simulink model "Full_Car_Model"  (R2023b)
settings: Solver=FixedStepAuto  StartTime=0.0  StopTime=t_end_sim  FixedStep=Ts_sim  RelTol=1e-3
values from neighbouring files (symbols this model uses):
  a_b_ref_sat = [ zeros(1,10) ... (first row only)    [A1_Init.m]    (also in C1_MonteCarloAnalysis.m)
  adaptive = 3    [A1_Init.m]    (also in C1_MonteCarloAnalysis.m = 1)
  data = A2_Full_car_model_parameters_4onBoard()    [A1_Init.m]    (also in C1_MonteCarloAnalysis.m)
  Ft_demand_F = [zeros(1,601) 200*ones(1,2400)]./data.R_F    [A1_Init.m]    (also in C1_MonteCarloAnalysis.m)
  Ft_demand_R = [zeros(1,(601-length(l_discr)))              200*ones(1,(2400+length(l_discr)))]./data.R_R    [A1_Init.m]    (also in C1_MonteCarloAnalysis.m)
  handmade_front = strcat(currentPath,'\Road_profiles\height_crg_files\','handmade_step_3cm_singlefunctions.crg')    [A1_Init.m]    (also in C1_MonteCarloAnalysis.m)
  handmade_mu_front = strcat(currentPath,'\Road_profiles\friction_crg_files\','handmade_fric_step_01_singlefunctions.crg')    [A1_Init.m]    (also in C1_MonteCarloAnalysis.m)
  handmade_mu_rear = handmade_mu_front    [A1_Init.m]    (also in C1_MonteCarloAnalysis.m)
  handmade_rear = handmade_front    [A1_Init.m]    (also in C1_MonteCarloAnalysis.m)
  LowLim_Q1 = -10    [A1_Init.m]    (also in C1_MonteCarloAnalysis.m)
  M = N    (= 10)    [A1_Init.m]    (also in C1_MonteCarloAnalysis.m)
  mu_distance = test_distance    [A1_Init.m]    (also in C1_MonteCarloAnalysis.m)
  mu_road = [ones(1,1001), 0.1*ones(1,2000)]    [A1_Init.m]    (also in C1_MonteCarloAnalysis.m)
  N = 10    [A1_Init.m]    (also in C1_MonteCarloAnalysis.m)
  N_iter = 3    [A1_Init.m]    (also in C1_MonteCarloAnalysis.m)
  omega_ini_F_L = x_u_dot_ini_F_L/data.R_F    [A1_Init.m]    (also in C1_MonteCarloAnalysis.m)
  omega_ini_F_R = x_u_dot_ini_R_R/data.R_F    [A1_Init.m]    (also in C1_MonteCarloAnalysis.m)
  omega_ini_R_L = x_u_dot_ini_R_L/data.R_R +2.483*1e-6    [A1_Init.m]    (also in C1_MonteCarloAnalysis.m)
  omega_ini_R_R = x_u_dot_ini_R_R/data.R_R+2.483*1e-6    [A1_Init.m]    (also in C1_MonteCarloAnalysis.m)
  passive = 2    [A1_Init.m]    (also in C1_MonteCarloAnalysis.m)
  Pitch = 0    [A1_Init.m]    (also in C1_MonteCarloAnalysis.m)
  Pitch_dot = 0    [A1_Init.m]    (also in C1_MonteCarloAnalysis.m)
  preview = 2    [A1_Init.m]    (also in C1_MonteCarloAnalysis.m)
  Q1 = 1e6    (= 1000000)    [A1_Init.m]    (also in C1_MonteCarloAnalysis.m)
  Q1_sat = 0    [A1_Init.m]    (also in C1_MonteCarloAnalysis.m)
  Q2 = 1e5    (= 100000)    [A1_Init.m]    (also in C1_MonteCarloAnalysis.m)
  QN1 = 0    [A1_Init.m]    (also in C1_MonteCarloAnalysis.m)
  QN2 = 0    [A1_Init.m]    (also in C1_MonteCarloAnalysis.m)
  R1 = 1e10    (= 10000000000)    [A1_Init.m]    (also in C1_MonteCarloAnalysis.m)
  r1_h0 = 0.99    [A1_Init.m]    (also in C1_MonteCarloAnalysis.m)
  r1_k = 1000    [A1_Init.m]    (also in C1_MonteCarloAnalysis.m)
  r1_max = 11    [A1_Init.m]    (also in C1_MonteCarloAnalysis.m)
  r1_min = -10    [A1_Init.m]    (also in C1_MonteCarloAnalysis.m)
  r2 = 2    [A1_Init.m]    (also in C1_MonteCarloAnalysis.m)
  R2 = 1e2    (= 100)    [A1_Init.m]    (also in C1_MonteCarloAnalysis.m)
  R2_rl = 2    [A1_Init.m]    (also in C1_MonteCarloAnalysis.m)
  road_profile = [zeros(1,801),ones(1,2200)*10*Step_selector]    [A1_Init.m]    (also in C1_MonteCarloAnalysis.m)
  T_distance = test_distance    [A1_Init.m]    (also in C1_MonteCarloAnalysis.m)
  T_hs_ini_F_L = 0    [A1_Init.m]    (also in C1_MonteCarloAnalysis.m)
  T_hs_ini_F_R = 0    [A1_Init.m]    (also in C1_MonteCarloAnalysis.m)
  T_hs_ini_R_L = 0    [A1_Init.m]    (also in C1_MonteCarloAnalysis.m)
  T_hs_ini_R_R = 0    [A1_Init.m]    (also in C1_MonteCarloAnalysis.m)
  test_distance = 0:0.01:30    [A1_Init.m]    (also in C1_MonteCarloAnalysis.m)
  theta_s_ini_F_L = 0    [A1_Init.m]    (also in C1_MonteCarloAnalysis.m)
  theta_s_ini_F_R = 0    [A1_Init.m]    (also in C1_MonteCarloAnalysis.m)
  theta_s_ini_R_L = 0    [A1_Init.m]    (also in C1_MonteCarloAnalysis.m)
  theta_s_ini_R_R = 0    [A1_Init.m]    (also in C1_MonteCarloAnalysis.m)
  theta_w_ini_F_L = -1.056*1e-2    (= -0.01056)    [A1_Init.m]    (also in C1_MonteCarloAnalysis.m)
  theta_w_ini_R_L = -1.056*1e-2    (= -0.01056)    [A1_Init.m]    (also in C1_MonteCarloAnalysis.m)
  Ts = 1e-3*[0 5 10 15 20 25 30 40 60 80 100]    [A1_Init.m]    (also in C1_MonteCarloAnalysis.m)
  w1_h0 = 0.0008    [A1_Init.m]    (also in C1_MonteCarloAnalysis.m)
  w1_k = 5000    [A1_Init.m]    (also in C1_MonteCarloAnalysis.m)
  w1_max = 9    [A1_Init.m]    (also in C1_MonteCarloAnalysis.m)
  w1_min = -10    [A1_Init.m]    (also in C1_MonteCarloAnalysis.m)
  w1_sat = 0.085    [A1_Init.m]    (also in C1_MonteCarloAnalysis.m)
  w2_h0 = 2    [A1_Init.m]    (also in C1_MonteCarloAnalysis.m)
  w2_inc = 0.05    [A1_Init.m]    (also in C1_MonteCarloAnalysis.m)
  w2_k = 10    [A1_Init.m]    (also in C1_MonteCarloAnalysis.m)
  w2_max = 5.3    [A1_Init.m]    (also in C1_MonteCarloAnalysis.m)
  w2_min = -10    [A1_Init.m]    (also in C1_MonteCarloAnalysis.m)
  Wmat_NMPC_init = [W(1,:) W(2,:) W(3,:) W(4,:)]    [A1_Init.m]    (also in C1_MonteCarloAnalysis.m)
  WNmat_NMPC_init = [WN(1,:) WN(2,:)]    [A1_Init.m]    (also in C1_MonteCarloAnalysis.m)
  X_0 = [z_b_dot_ini z_b_ini z_u_dot_ini_F_L z_u_ini_F_L x_b_dot_ini x_b_ini x_u_dot_ini_F_L x_u_ini_F_L          omega_ini_F_L theta_w_ini_F_L omega_ini_F_L theta_s_ini_F_L torque_ini_F_L]    [A1_Init.m]    (also in C1_MonteCarloAnalysis.m)
  x_b_dot_ini = speed_ini/3.6    (= 11.1111111111)    [A1_Init.m]    (also in C1_MonteCarloAnalysis.m)
  x_b_ini = data.b+pos_ini    [A1_Init.m]    (also in C1_MonteCarloAnalysis.m)
  x_u_dot_ini_F_L = speed_ini/3.6 - 1.125*1e-4    (= 11.1109986111)    [A1_Init.m]    (also in C1_MonteCarloAnalysis.m)
  x_u_dot_ini_F_R = speed_ini/3.6 - 1.125*1e-4    (= 11.1109986111)    [A1_Init.m]    (also in C1_MonteCarloAnalysis.m)
  x_u_dot_ini_R_L = speed_ini/3.6 - 1.125*1e-4    (= 11.1109986111)    [A1_Init.m]    (also in C1_MonteCarloAnalysis.m)
  x_u_dot_ini_R_R = speed_ini/3.6 - 1.125*1e-4    (= 11.1109986111)    [A1_Init.m]    (also in C1_MonteCarloAnalysis.m)
  x_u_ini_F_L = data.a+data.b+pos_ini    [A1_Init.m]    (also in C1_MonteCarloAnalysis.m)
  x_u_ini_F_R = data.a+data.b+pos_ini    [A1_Init.m]    (also in C1_MonteCarloAnalysis.m)
  x_u_ini_R_L = pos_ini    (= 0)    [A1_Init.m]    (also in C1_MonteCarloAnalysis.m)
  x_u_ini_R_R = pos_ini    (= 0)    [A1_Init.m]    (also in C1_MonteCarloAnalysis.m)
  z_b_dot_ini = 0    [A1_Init.m]    (also in C1_MonteCarloAnalysis.m)
  z_b_ini = 0    [A1_Init.m]    (also in C1_MonteCarloAnalysis.m)
  z_u_dot_ini_F_L = 0    [A1_Init.m]    (also in C1_MonteCarloAnalysis.m)
  z_u_dot_ini_F_R = 0    [A1_Init.m]    (also in C1_MonteCarloAnalysis.m)
  z_u_dot_ini_R_L = 0    [A1_Init.m]    (also in C1_MonteCarloAnalysis.m)
  z_u_dot_ini_R_R = 0    [A1_Init.m]    (also in C1_MonteCarloAnalysis.m)
  z_u_ini_F_L = 0    [A1_Init.m]    (also in C1_MonteCarloAnalysis.m)
  z_u_ini_F_R = 0    [A1_Init.m]    (also in C1_MonteCarloAnalysis.m)
  z_u_ini_R_L = 0    [A1_Init.m]    (also in C1_MonteCarloAnalysis.m)
  z_u_ini_R_R = 0    [A1_Init.m]    (also in C1_MonteCarloAnalysis.m)
undefined symbols (not defined in the file or in its folder): Delay_step, road_with_noise
libraries: mfswift_library x8, rllib x4, simulink x4
(part 1 of 7)
settings Model: Creator=victor  LastModifiedBy=d106370
settings SolverCC: AlgebraicLoopSolver=TrustRegion
settings DataIOCC: SaveOutput=off  SignalLogging=off  DSMLogging=off  SaveTime=off  ReturnWorkspaceOutputs=off
settings DebuggingCC: UnconnectedInputMsg=warning  UnconnectedOutputMsg=warning  UnconnectedLineMsg=warning
settings ModelReferenceCC: EnableRefExpFcnMdlSchedulingChecks=on
settings SFSimCC: CustomCodeUndefinedFunction=UseInterfaceOnly
settings RTWCC: DLArmComputeVersion=19.05

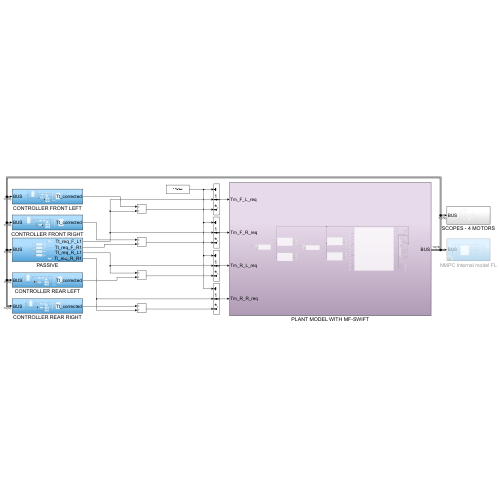
[thumbnail: Simulink's stored preview of the top-level diagram]
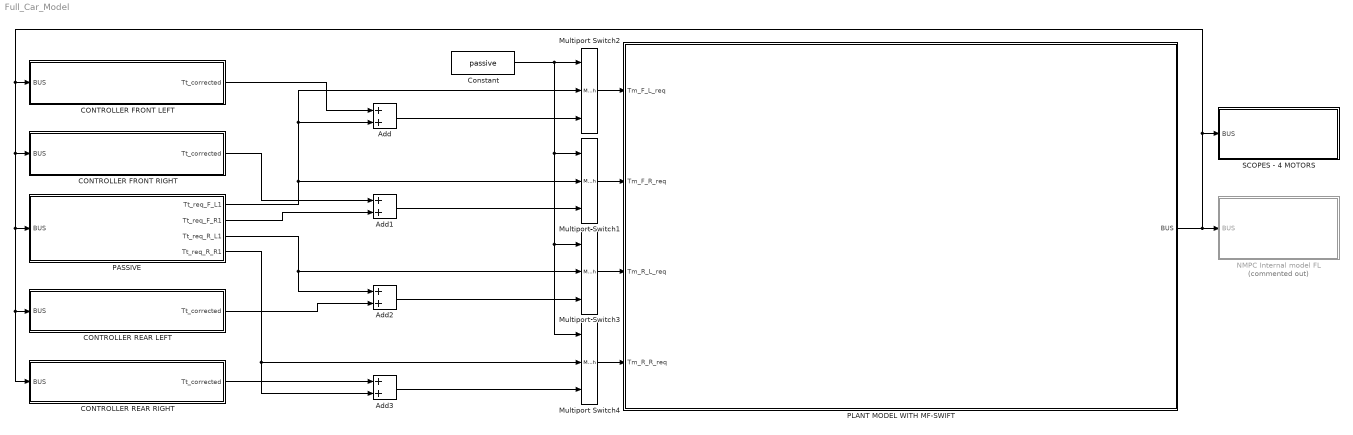
== system Full_Car_Model ==
  Add{,1..3} (4 alike) : Sum
  CONTROLLER FRONT LEFT : Subsystem
  CONTROLLER FRONT RIGHT : Subsystem
  CONTROLLER REAR LEFT : Subsystem
  CONTROLLER REAR RIGHT : Subsystem
  Constant : Constant  Value=passive
  Multiport Switch{1..4} (4 alike) : MultiPortSwitch  Inputs=2  SaturateOnIntegerOverflow=off  InputSameDT=off
  NMPC Internal model FL : Subsystem  Commented=on
  PASSIVE : Subsystem
  PLANT MODEL WITH MF-SWIFT : Subsystem
  SCOPES - 4 MOTORS : Subsystem
  wires:
  Add3/1 -> Multiport Switch4/3
  Multiport Switch4/1 -> PLANT MODEL WITH MF-SWIFT/4(Tm_R_R_req)
  Multiport Switch2/1 -> PLANT MODEL WITH MF-SWIFT/1(Tm_F_L_req)
  CONTROLLER REAR LEFT/1(Tt_corrected) -> Add2/2
  Multiport Switch1/1 -> PLANT MODEL WITH MF-SWIFT/2(Tm_F_R_req)
  PASSIVE/2(Tt_req_F_R1) -> Add1/2
  CONTROLLER FRONT RIGHT/1(Tt_corrected) -> Add1/1
  CONTROLLER FRONT LEFT/1(Tt_corrected) -> Add/1
  PASSIVE/1(Tt_req_F_L1) -> Multiport Switch1/2, Multiport Switch2/2, Add/2
  Add2/1 -> Multiport Switch3/3
  Add/1 -> Multiport Switch2/3
  PLANT MODEL WITH MF-SWIFT/1(BUS) -> CONTROLLER FRONT LEFT/1(BUS), CONTROLLER REAR RIGHT/1(BUS), CONTROLLER REAR LEFT/1(BUS), PASSIVE/1(BUS), CONTROLLER FRONT RIGHT/1(BUS), SCOPES - 4 MOTORS/1(BUS), NMPC Internal model FL/1(BUS)
  Add1/1 -> Multiport Switch1/3
  CONTROLLER REAR RIGHT/1(Tt_corrected) -> Add3/1
  PASSIVE/3(Tt_req_R_L1) -> Add2/1, Multiport Switch3/2
  Constant/1 -> Multiport Switch4/1, Multiport Switch3/1, Multiport Switch1/1, Multiport Switch2/1
  Multiport Switch3/1 -> PLANT MODEL WITH MF-SWIFT/3(Tm_R_L_req)
  PASSIVE/4(Tt_req_R_R1) -> Multiport Switch4/2, Add3/2

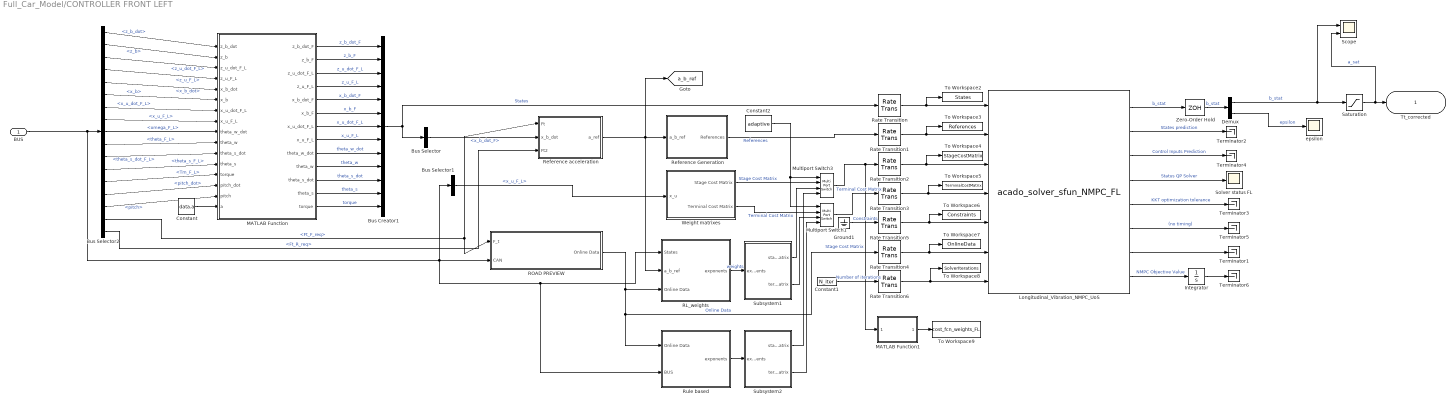
== system Full_Car_Model/CONTROLLER FRONT LEFT ==
  BUS : Inport
  Bus Creator1 : BusCreator  Inputs=13
  Bus Selector : BusSelector  OutputSignals=x_b_dot_F
  Bus Selector1 : BusSelector  OutputSignals=States.x_u_F_L
  Bus Selector2 : BusSelector  OutputSignals=States.z_b_dot,States.z_b,States.z_u_dot_F_L,States.z_u_F_L,States.x_b_dot,States.x_b,States.x_u_dot_F_L,States.x_u_F_L,States.omega_F_L,States.theta_F_L,Differentials.theta_s_dot_F_L,Differentials.theta_s_F_L,Traction_forces.Tm_F_L,States.pitch_dot,States.pitch,Traction_forces.Ft_F_req,Traction_forces.Ft_R_req
  Constant : Constant  Value=data.a
  Constant1 : Constant  Value=N_iter
  Constant2 : Constant  Value=adaptive
  Demux : Demux  Outputs=2
  Ground1 : Ground
  Integrator : Integrator
  Longitudinal_Vibration_NMPC_UoS : S-Function  FunctionName=acado_solver_sfun_NMPC_FL  Parameters=xInit, zInit, uInit, Wmat_NMPC_init, WNmat_NMPC_init, bValues  SFunctionDeploymentMode=off  EnableBusSupport=off  mask(Legacy Function){SFunctionSpec=acado_step(ACADOinput u1[1], ACADOoutput y1[1]), ShowSpec=on}
      mask prompts: ShowSpec "Display function specification"
      mask help:
      | This block allows you to call the legacy functions specified by the following Legacy Code Tool definition:
      | def.SFunctionName = 'acado_solver_sfun';
      | def.OutputFcnSpec = 'acado_step(ACADOinput u1[1], ACADOoutput y1[1])';
      | def.StartFcnSpec = 'acado_initialize( void )';
      | def.TerminateFcnSpec = 'acado_cleanup( void )';
      | def.HeaderFiles = {'acado_common.h', 'acado_solver_sfunction.h'};
      | def.SourceFiles = {'acado_solver.c', 'acado_integrator.c', 'acado_auxiliary_functions.c', 'acado_solver_sfunction.c', 'acado_qpoases_interface.cpp', 'qpoases/SRC/Bounds.cpp', 'qpoases/SRC/Constraints.cpp', 'qpoases/SRC/CyclingManager.cpp', 'qpoases/SRC/Indexlist.cpp', 'qpoases/SRC/MessageHandling.cpp', 'qpoases/SRC/QProblem.cpp', 'qpoases/SRC/QProblemB.cpp', 'qpoases/SRC/SubjectTo.cpp', 'qpoases/SRC/Utils.cpp', 'qpoases/SRC/EXTRAS/SolutionAnalysis.cpp'};
      | def.IncPaths = {'qpoases', 'qpoases/INCLUDE', 'qpoases/SRC'};
      | def.Options.language = 'C++';
      mask Help: <p>This block was generated automatically by the Legacy Code Tool. For detailed help on this tool, call<a href="matlab:legacy_code('help')"> legacy_code('help')</a>.</p>
      mask Callback ShowSpec:
      | if strcmp(get_param(gcbh, 'ShowSpec'), 'on')
      |   set_param(gcbh, 'MaskDisplay', sprintf('fprintf(''%s'');', get_param(gcbh, 'SFunctionSpec')));
      | else
      |   set_param(gcbh, 'MaskDisplay', sprintf('fprintf(''%s'');', get_param(gcbh, 'FunctionName')));
      | end
      mask Display: fprintf('acado_step(ACADOinput u1[1], ACADOoutput y1[1])');
  MATLAB Function : MATLAB Function  TreatAsAtomicUnit=on
  MATLAB Function1 : MATLAB Function  TreatAsAtomicUnit=on
  Multiport Switch1 : MultiPortSwitch  SaturateOnIntegerOverflow=off  InputSameDT=off
  Multiport Switch3 : MultiPortSwitch  SaturateOnIntegerOverflow=off  InputSameDT=off
  RL_weights : Subsystem
  ROAD PREVIEW : Subsystem
  Rate Transition : RateTransition  InitialCondition=X_0  OutPortSampleTime=Ts(2)
  Rate Transition{1,4..6} (4 alike) : RateTransition  OutPortSampleTime=Ts(2)
  Rate Transition2 : RateTransition  InitialCondition=Wmat_NMPC_init  OutPortSampleTime=Ts(2)
  Rate Transition3 : RateTransition  InitialCondition=WNmat_NMPC_init  OutPortSampleTime=Ts(2)
  Reference Generation : MATLAB Function  TreatAsAtomicUnit=on
  Reference acceleration : Subsystem
  Rule based : Subsystem
  Saturation : Saturate  UpperLimit=data.Ub_Tm  LowerLimit=data.Lb_Tm
  Scope : Scope  NumInputPorts=2
  Solver status FL : Scope
  Subsystem1 : Subsystem
  Subsystem2 : Subsystem
  Terminator{1..6} (6 alike) : Terminator
  To Workspace2 : ToWorkspace  VariableName=States  SaveFormat=Timeseries  SampleTime=-1
  To Workspace3 : ToWorkspace  VariableName=References  SaveFormat=Timeseries  SampleTime=-1
  To Workspace4 : ToWorkspace  VariableName=StageCostMatrix  SaveFormat=Timeseries  SampleTime=-1
  To Workspace5 : ToWorkspace  VariableName=TerminalCostMatrix  SaveFormat=Timeseries  SampleTime=-1
  To Workspace6 : ToWorkspace  VariableName=Constraints  SaveFormat=Timeseries  SampleTime=-1
  To Workspace7 : ToWorkspace  VariableName=OnlineData  SaveFormat=Timeseries  SampleTime=-1
  To Workspace8 : ToWorkspace  VariableName=SolverIterations  SaveFormat=Timeseries  SampleTime=-1
  To Workspace9 : ToWorkspace  VariableName=cost_fcn_weights_FL  SaveFormat=Timeseries  SampleTime=-1
  Weight matrixes : Subsystem
  Zero-Order Hold : ZeroOrderHold  SampleTime=Ts(2)
  epsilon : Scope
  Tt_corrected : Outport
  tag scope: a_b_ref=global
  wires:
  Subsystem1/2(terminal cost matrix) -> Multiport Switch1/3
  Saturation/1 -> Scope/2, Tt_corrected/1  "a_sat"
  MATLAB Function/8(x_u_F_L) -> Bus Creator1/8  "x_u_F_L"
  MATLAB Function/3(z_u_dot_F_L) -> Bus Creator1/3  "z_u_dot_F_L"
  Weight matrixes/1(Stage Cost Matrix) -> Multiport Switch3/2  "Stage Cost Matrix"
  MATLAB Function/1(z_b_dot_F) -> Bus Creator1/1  "z_b_dot_F"
  Constant1/1 -> Rate Transition6/1  "Number of iterations"
  MATLAB Function/2(z_b_F) -> Bus Creator1/2  "z_b_F"
  MATLAB Function/6(x_b_F) -> Bus Creator1/6  "x_b_F"
  Bus Selector2/14 -> MATLAB Function/14(pitch_dot)  "<pitch_dot>"
  MATLAB Function/7(x_u_dot_F_L) -> Bus Creator1/7  "x_u_dot_F_L"
  Longitudinal_Vibration_NMPC_UoS/2 -> Terminator2/1  "States prediction"
  Weight matrixes/2(Terminal Cost Matrix) -> Multiport Switch1/2  "Terminal Cost Matrix"
  Bus Selector2/6 -> MATLAB Function/6(x_b)  "<x_b>"
  Longitudinal_Vibration_NMPC_UoS/4 -> Solver status FL/1  "Status QP Solver"
  Reference acceleration/1(a_ref) -> Reference Generation/1(a_b_ref), [a_b_ref], RL_weights/2(a_b_ref)
  Integrator/1 -> Terminator6/1
  Bus Selector2/1 -> MATLAB Function/1(z_b_dot)  "<z_b_dot>"
  Rate Transition2/1 -> Longitudinal_Vibration_NMPC_UoS/3, To Workspace4/1
  Bus Selector2/9 -> MATLAB Function/9("theta_w_dot ")  "<omega_F_L>"
  Rate Transition4/1 -> Longitudinal_Vibration_NMPC_UoS/6, To Workspace7/1
  Bus Selector2/8 -> MATLAB Function/8("x_u_F_L ")  "<x_u_F_L>"
  BUS/1 -> Bus Selector2/1, Rule based/2(BUS), RL_weights/1(States), Bus Selector1/1, ROAD PREVIEW/2(CAN)
  Rate Transition3/1 -> Longitudinal_Vibration_NMPC_UoS/4, To Workspace5/1
  RL_weights/1(exponents) -> Subsystem1/1(exponents)  "weights"
  ROAD PREVIEW/1(Online Data) -> Rule based/1(Online Data), Rate Transition4/1, RL_weights/3(Online Data)  "Online Data"
  Bus Selector2/12 -> MATLAB Function/12("theta_s ")  "<theta_s_F_L>"
  Subsystem2/2(terminal cost matrix) -> Multiport Switch1/4
  MATLAB Function/9(theta_w_dot) -> Bus Creator1/9  "theta_w_dot"
  Multiport Switch3/1 -> Rate Transition2/1, MATLAB Function1/1(Wmat_NMPC)  "Stage Cost Matrix"
  Constant/1 -> MATLAB Function/16(a)
  Bus Selector2/2 -> MATLAB Function/2(z_b)  "<z_b>"
  Bus Selector2/11 -> MATLAB Function/11("theta_s_dot ")  "<theta_s_dot_F_L>"
  MATLAB Function/13(torque) -> Bus Creator1/13  "torque"
  Longitudinal_Vibration_NMPC_UoS/3 -> Terminator4/1  "Control Inputs Prediction"
  MATLAB Function/10(theta_w) -> Bus Creator1/10  "theta_w"
  Longitudinal_Vibration_NMPC_UoS/6 -> Terminator5/1  "(no timing)"
  Demux/2 -> epsilon/1  "epsilon"
  Rate Transition5/1 -> Longitudinal_Vibration_NMPC_UoS/5, To Workspace6/1
  MATLAB Function/11(theta_s_dot) -> Bus Creator1/11  "theta_s_dot"
  MATLAB Function/5(x_b_dot_F) -> Bus Creator1/5  "x_b_dot_F"
  Bus Selector/1 -> Reference acceleration/2(x_b_dot)  "<x_b_dot_F>"
  Longitudinal_Vibration_NMPC_UoS/7 -> Terminator1/1
  Bus Selector2/13 -> MATLAB Function/13("torque ")  "<Tm_F_L>"
  Bus Selector2/16 -> Reference acceleration/1(Ft), ROAD PREVIEW/1(F_t)  "<Ft_F_req>"
  Subsystem1/1(stage cost matrix) -> Multiport Switch3/3
  Bus Selector2/10 -> MATLAB Function/10("theta_w ")  "<theta_F_L>"
  Reference Generation/1(References) -> Rate Transition1/1  "References"
  Ground1/1 -> Rate Transition5/1  "Constraints"
  Rate Transition6/1 -> Longitudinal_Vibration_NMPC_UoS/7, To Workspace8/1
  Subsystem2/1(stage cost matrix) -> Multiport Switch3/4
  Bus Selector2/5 -> MATLAB Function/5(x_b_dot)  "<x_b_dot>"
  Bus Selector2/7 -> MATLAB Function/7("x_u_dot_F_L ")  "<x_u_dot_F_L>"
  Bus Selector2/15 -> MATLAB Function/15(pitch)  "<pitch>"
  MATLAB Function/12(theta_s) -> Bus Creator1/12  "theta_s"
  Longitudinal_Vibration_NMPC_UoS/5 -> Terminator3/1  "KKT optimization tolerance"
  Bus Creator1/1 -> Rate Transition/1, Bus Selector/1  "States"
  Rate Transition/1 -> Longitudinal_Vibration_NMPC_UoS/1, To Workspace2/1
  Bus Selector2/4 -> MATLAB Function/4("z_u_F_L ")  "<z_u_F_L>"
  Bus Selector2/17 -> Reference acceleration/3(Ft2)  "<Ft_R_req>"
  MATLAB Function/4(z_u_F_L) -> Bus Creator1/4  "z_u_F_L"
  Rate Transition1/1 -> Longitudinal_Vibration_NMPC_UoS/2, To Workspace3/1
  Multiport Switch1/1 -> Rate Transition3/1  "Terminal Cost Matrix"
  Bus Selector1/1 -> Weight matrixes/1(x_u)  "<x_u_F_L>"
  Bus Selector2/3 -> MATLAB Function/3("z_u_dot_F_L ")  "<z_u_dot_F_L>"
  Constant2/1 -> Multiport Switch3/1, Multiport Switch1/1
  Longitudinal_Vibration_NMPC_UoS/8 -> Integrator/1  "NMPC Objective Value"
  Longitudinal_Vibration_NMPC_UoS/1 -> Zero-Order Hold/1  "b_stat"
  Demux/1 -> Scope/1, Saturation/1  "b_stat"
  Zero-Order Hold/1 -> Demux/1  "b_stat"
  MATLAB Function1/1(cost_fcn_weights) -> To Workspace9/1
  Rule based/1(exponents) -> Subsystem2/1(exponents)

== system Full_Car_Model/CONTROLLER FRONT RIGHT ==
  BUS : Inport
  Bus Creator1 : BusCreator  Inputs=13
  Bus Selector : BusSelector  OutputSignals=x_b_dot_F
  Bus Selector1 : BusSelector  OutputSignals=States.x_u_F_R
  Bus Selector2 : BusSelector  OutputSignals=States.z_b_dot,States.z_b,States.z_u_dot_F_R,States.z_u_F_R,States.x_b_dot,States.x_b,States.x_u_dot_F_R,States.x_u_F_R,States.omega_F_R,States.theta_F_R,Differentials.theta_s_dot_F_R,Differentials.theta_s_F_R,Traction_forces.Tm_F_R,States.pitch_dot,States.pitch,Traction_forces.Ft_F_req,Traction_forces.Ft_R_req
  Constant : Constant  Value=data.a
  Constant1 : Constant  Value=N_iter
  Constant2 : Constant  Value=adaptive
  Demux : Demux  Outputs=2
  Ground1 : Ground
  Integrator : Integrator
  Longitudinal_Vibration_NMPC_UoS : S-Function  FunctionName=acado_solver_sfun_NMPC_FR  Parameters=xInit, zInit, uInit, Wmat_NMPC_init, WNmat_NMPC_init, bValues  SFunctionDeploymentMode=off  EnableBusSupport=off  mask(Legacy Function){SFunctionSpec=acado_step(ACADOinput u1[1], ACADOoutput y1[1]), ShowSpec=on}
      mask prompts: ShowSpec "Display function specification"
      mask help:
      | This block allows you to call the legacy functions specified by the following Legacy Code Tool definition:
      | def.SFunctionName = 'acado_solver_sfun';
      | def.OutputFcnSpec = 'acado_step(ACADOinput u1[1], ACADOoutput y1[1])';
      | def.StartFcnSpec = 'acado_initialize( void )';
      | def.TerminateFcnSpec = 'acado_cleanup( void )';
      | def.HeaderFiles = {'acado_common.h', 'acado_solver_sfunction.h'};
      | def.SourceFiles = {'acado_solver.c', 'acado_integrator.c', 'acado_auxiliary_functions.c', 'acado_solver_sfunction.c', 'acado_qpoases_interface.cpp', 'qpoases/SRC/Bounds.cpp', 'qpoases/SRC/Constraints.cpp', 'qpoases/SRC/CyclingManager.cpp', 'qpoases/SRC/Indexlist.cpp', 'qpoases/SRC/MessageHandling.cpp', 'qpoases/SRC/QProblem.cpp', 'qpoases/SRC/QProblemB.cpp', 'qpoases/SRC/SubjectTo.cpp', 'qpoases/SRC/Utils.cpp', 'qpoases/SRC/EXTRAS/SolutionAnalysis.cpp'};
      | def.IncPaths = {'qpoases', 'qpoases/INCLUDE', 'qpoases/SRC'};
      | def.Options.language = 'C++';
      mask Help: <p>This block was generated automatically by the Legacy Code Tool. For detailed help on this tool, call<a href="matlab:legacy_code('help')"> legacy_code('help')</a>.</p>
      mask Callback ShowSpec:
      | if strcmp(get_param(gcbh, 'ShowSpec'), 'on')
      |   set_param(gcbh, 'MaskDisplay', sprintf('fprintf(''%s'');', get_param(gcbh, 'SFunctionSpec')));
      | else
      |   set_param(gcbh, 'MaskDisplay', sprintf('fprintf(''%s'');', get_param(gcbh, 'FunctionName')));
      | end
      mask Display: fprintf('acado_step(ACADOinput u1[1], ACADOoutput y1[1])');
  MATLAB Function : MATLAB Function  TreatAsAtomicUnit=on
  Multiport Switch1 : MultiPortSwitch  SaturateOnIntegerOverflow=off  InputSameDT=off
  Multiport Switch3 : MultiPortSwitch  SaturateOnIntegerOverflow=off  InputSameDT=off
  RL_weights : Subsystem
  ROAD PREVIEW : Subsystem
  Rate Transition : RateTransition  InitialCondition=X_0  OutPortSampleTime=Ts(2)
  Rate Transition{1,4..6} (4 alike) : RateTransition  OutPortSampleTime=Ts(2)
  Rate Transition2 : RateTransition  InitialCondition=Wmat_NMPC_init  OutPortSampleTime=Ts(2)
  Rate Transition3 : RateTransition  InitialCondition=WNmat_NMPC_init  OutPortSampleTime=Ts(2)
  Reference Generation : MATLAB Function  TreatAsAtomicUnit=on
  Reference acceleration : Subsystem
  Rule based : Subsystem
  Saturation : Saturate  UpperLimit=data.Ub_Tm  LowerLimit=data.Lb_Tm
  Subsystem1 : Subsystem
  Subsystem2 : Subsystem
  Terminator{1..8} (8 alike) : Terminator
  Weight matrixes : Subsystem
  Zero-Order Hold : ZeroOrderHold  SampleTime=Ts(2)
  Tt_corrected : Outport
  wires:
  Bus Selector2/7 -> MATLAB Function/7("x_u_dot_F_R ")  "<x_u_dot_F_R>"
  Weight matrixes/2(Terminal Cost Matrix) -> Multiport Switch1/2  "Terminal Cost Matrix"
  MATLAB Function/5(x_b_dot_F) -> Bus Creator1/5  "x_b_dot_F"
  ROAD PREVIEW/1(Online Data) -> Rule based/1(Online Data), Rate Transition4/1, RL_weights/2(Online Data)  "Online Data"
  Subsystem2/1(stage cost matrix) -> Multiport Switch3/4
  Bus Selector2/11 -> MATLAB Function/11("theta_s_dot ")  "<theta_s_dot_F_R>"
  Multiport Switch3/1 -> Rate Transition2/1  "Stage Cost Matrix"
  Longitudinal_Vibration_NMPC_UoS/4 -> Terminator2/1  "Status QP Solver"
  MATLAB Function/2(z_b_F) -> Bus Creator1/2  "z_b_F"
  Bus Selector2/3 -> MATLAB Function/3("z_u_dot_F_R ")  "<z_u_dot_F_R>"
  Rule based/1(exponents) -> Subsystem2/1(exponents)
  Subsystem2/2(terminal cost matrix) -> Multiport Switch1/4
  MATLAB Function/10(theta_w) -> Bus Creator1/10  "theta_w"
  Integrator/1 -> Terminator7/1
  Longitudinal_Vibration_NMPC_UoS/6 -> Terminator4/1  "(no timing)"
  Longitudinal_Vibration_NMPC_UoS/3 -> Terminator5/1  "Control Inputs Prediction"
  MATLAB Function/7(x_u_dot_F_R) -> Bus Creator1/7  "x_u_dot_F_R"
  Bus Selector2/14 -> MATLAB Function/14(pitch_dot)  "<pitch_dot>"
  MATLAB Function/11(theta_s_dot) -> Bus Creator1/11  "theta_s_dot"
  Rate Transition6/1 -> Longitudinal_Vibration_NMPC_UoS/7
  Multiport Switch1/1 -> Rate Transition3/1  "Terminal Cost Matrix"
  MATLAB Function/3(z_u_dot_F_R) -> Bus Creator1/3  "z_u_dot_F_R"
  Bus Selector2/6 -> MATLAB Function/6(x_b)  "<x_b>"
  Constant2/1 -> Multiport Switch1/1, Multiport Switch3/1
  Constant1/1 -> Rate Transition6/1  "Number of iterations"
  Rate Transition5/1 -> Longitudinal_Vibration_NMPC_UoS/5
  Demux/2 -> Terminator8/1  "epsilon"
  Bus Selector2/15 -> MATLAB Function/15(pitch)  "<pitch>"
  Bus Selector2/17 -> Reference acceleration/3(Ft2)  "<Ft_R_req>"
  MATLAB Function/13(torque) -> Bus Creator1/13  "torque"
  Bus Selector2/9 -> MATLAB Function/9("theta_w_dot ")  "<omega_F_R>"
  RL_weights/1(exponents) -> Subsystem1/1(exponents)
  Bus Selector2/4 -> MATLAB Function/4("z_u_F_R ")  "<z_u_F_R>"
  Weight matrixes/1(Stage Cost Matrix) -> Multiport Switch3/2  "Stage Cost Matrix"
  Ground1/1 -> Rate Transition5/1  "Constraints"
  MATLAB Function/12(theta_s) -> Bus Creator1/12  "theta_s"
  Rate Transition/1 -> Longitudinal_Vibration_NMPC_UoS/1
  MATLAB Function/9(theta_w_dot) -> Bus Creator1/9  "theta_w_dot"
  Bus Selector2/2 -> MATLAB Function/2(z_b)  "<z_b>"
  Bus Selector2/16 -> Reference acceleration/1(Ft), ROAD PREVIEW/1(F_t)  "<Ft_F_req>"
  MATLAB Function/6(x_b_F) -> Bus Creator1/6  "x_b_F"
  Constant/1 -> MATLAB Function/16(a)
  Rate Transition2/1 -> Longitudinal_Vibration_NMPC_UoS/3
  Bus Selector2/5 -> MATLAB Function/5(x_b_dot)  "<x_b_dot>"
  Bus Selector2/13 -> MATLAB Function/13("torque ")  "<Tm_F_R>"
  Bus Selector/1 -> Reference acceleration/2(x_b_dot)  "<x_b_dot_F>"
  Bus Creator1/1 -> Rate Transition/1, Bus Selector/1  "States"
  Longitudinal_Vibration_NMPC_UoS/8 -> Integrator/1  "NMPC Objective Value"
  Longitudinal_Vibration_NMPC_UoS/5 -> Terminator3/1  "KKT optimization tolerance"
  MATLAB Function/1(z_b_dot_F) -> Bus Creator1/1  "z_b_dot_F"
  Bus Selector2/8 -> MATLAB Function/8("x_u_F_R ")  "<x_u_F_R>"
  Rate Transition3/1 -> Longitudinal_Vibration_NMPC_UoS/4
  Saturation/1 -> Tt_corrected/1
  Bus Selector2/12 -> MATLAB Function/12("theta_s ")  "<theta_s_F_R>"
  Bus Selector2/1 -> MATLAB Function/1(z_b_dot)  "<z_b_dot>"
  Bus Selector2/10 -> MATLAB Function/10("theta_w ")  "<theta_F_R>"
  MATLAB Function/8(x_u_F_R) -> Bus Creator1/8  "x_u_F_R"
  Subsystem1/2(terminal cost matrix) -> Multiport Switch1/3
  Subsystem1/1(stage cost matrix) -> Multiport Switch3/3
  Rate Transition1/1 -> Longitudinal_Vibration_NMPC_UoS/2
  Reference acceleration/1(a_ref) -> RL_weights/3(a_b_ref), Reference Generation/1(a_b_ref)
  Longitudinal_Vibration_NMPC_UoS/7 -> Terminator1/1
  BUS/1 -> RL_weights/1(States), Rule based/2(BUS), ROAD PREVIEW/2(CAN), Bus Selector1/1, Bus Selector2/1
  Rate Transition4/1 -> Longitudinal_Vibration_NMPC_UoS/6
  Longitudinal_Vibration_NMPC_UoS/2 -> Terminator6/1  "States prediction"
  MATLAB Function/4(z_u_F_R) -> Bus Creator1/4  "z_u_F_R"
  Zero-Order Hold/1 -> Demux/1
  Longitudinal_Vibration_NMPC_UoS/1 -> Zero-Order Hold/1  "First Control Input"
  Demux/1 -> Saturation/1
  Bus Selector1/1 -> Weight matrixes/1(x_u)  "<x_u_F_R>"
  Reference Generation/1(References) -> Rate Transition1/1  "References"

== system Full_Car_Model/CONTROLLER REAR LEFT ==
  BUS : Inport
  Bus Creator1 : BusCreator  Inputs=13
  Bus Selector : BusSelector  OutputSignals=x_b_dot_R
  Bus Selector1 : BusSelector  OutputSignals=States.x_u_R_L
  Bus Selector2 : BusSelector  OutputSignals=States.z_b_dot,States.z_b,States.z_u_dot_R_L,States.z_u_R_L,States.x_b_dot,States.x_b,States.x_u_dot_R_L,States.x_u_R_L,States.omega_R_L,States.theta_R_L,Differentials.theta_s_dot_R_L,Differentials.theta_s_R_L,Traction_forces.Tm_R_L,States.pitch_dot,States.pitch,Traction_forces.Ft_R_req,Traction_forces.Ft_F_req
  Constant : Constant  Value=data.b
  Constant1 : Constant  Value=N_iter
  Constant2 : Constant  Value=adaptive
  Demux : Demux  Outputs=2
  Ground1 : Ground
  Integrator : Integrator
  Longitudinal_Vibration_NMPC_UoS : S-Function  FunctionName=acado_solver_sfun_NMPC_RL  Parameters=xInit, zInit, uInit, Wmat_NMPC_init, WNmat_NMPC_init, bValues  SFunctionDeploymentMode=off  EnableBusSupport=off  mask(Legacy Function){SFunctionSpec=acado_step(ACADOinput u1[1], ACADOoutput y1[1]), ShowSpec=on}
      mask prompts: ShowSpec "Display function specification"
      mask help:
      | This block allows you to call the legacy functions specified by the following Legacy Code Tool definition:
      | def.SFunctionName = 'acado_solver_sfun';
      | def.OutputFcnSpec = 'acado_step(ACADOinput u1[1], ACADOoutput y1[1])';
      | def.StartFcnSpec = 'acado_initialize( void )';
      | def.TerminateFcnSpec = 'acado_cleanup( void )';
      | def.HeaderFiles = {'acado_common.h', 'acado_solver_sfunction.h'};
      | def.SourceFiles = {'acado_solver.c', 'acado_integrator.c', 'acado_auxiliary_functions.c', 'acado_solver_sfunction.c', 'acado_qpoases_interface.cpp', 'qpoases/SRC/Bounds.cpp', 'qpoases/SRC/Constraints.cpp', 'qpoases/SRC/CyclingManager.cpp', 'qpoases/SRC/Indexlist.cpp', 'qpoases/SRC/MessageHandling.cpp', 'qpoases/SRC/QProblem.cpp', 'qpoases/SRC/QProblemB.cpp', 'qpoases/SRC/SubjectTo.cpp', 'qpoases/SRC/Utils.cpp', 'qpoases/SRC/EXTRAS/SolutionAnalysis.cpp'};
      | def.IncPaths = {'qpoases', 'qpoases/INCLUDE', 'qpoases/SRC'};
      | def.Options.language = 'C++';
      mask Help: <p>This block was generated automatically by the Legacy Code Tool. For detailed help on this tool, call<a href="matlab:legacy_code('help')"> legacy_code('help')</a>.</p>
      mask Callback ShowSpec:
      | if strcmp(get_param(gcbh, 'ShowSpec'), 'on')
      |   set_param(gcbh, 'MaskDisplay', sprintf('fprintf(''%s'');', get_param(gcbh, 'SFunctionSpec')));
      | else
      |   set_param(gcbh, 'MaskDisplay', sprintf('fprintf(''%s'');', get_param(gcbh, 'FunctionName')));
      | end
      mask Display: fprintf('acado_step(ACADOinput u1[1], ACADOoutput y1[1])');
  MATLAB Function : MATLAB Function  TreatAsAtomicUnit=on
  MATLAB Function1 : MATLAB Function  TreatAsAtomicUnit=on
  Multiport Switch1 : MultiPortSwitch  SaturateOnIntegerOverflow=off  InputSameDT=off
  Multiport Switch3 : MultiPortSwitch  SaturateOnIntegerOverflow=off  InputSameDT=off
  RL_weights : Subsystem
  ROAD PREVIEW : Subsystem
  Rate Transition : RateTransition  InitialCondition=X_0  OutPortSampleTime=Ts(2)
  Rate Transition{1,4..6} (4 alike) : RateTransition  OutPortSampleTime=Ts(2)
  Rate Transition2 : RateTransition  InitialCondition=Wmat_NMPC_init  OutPortSampleTime=Ts(2)
  Rate Transition3 : RateTransition  InitialCondition=WNmat_NMPC_init  OutPortSampleTime=Ts(2)
  Reference Generation : MATLAB Function  TreatAsAtomicUnit=on
  Reference acceleration : Subsystem
  Rule based : Subsystem
  Saturation : Saturate  UpperLimit=data.Ub_Tm  LowerLimit=data.Lb_Tm
  Solver status RL : Scope
  Subsystem1 : Subsystem
  Subsystem2 : Subsystem
  Terminator{1..6} (6 alike) : Terminator
  To Workspace9 : ToWorkspace  VariableName=cost_fcn_weights_RL  SaveFormat=Timeseries  SampleTime=-1
  Weight matrixes : Subsystem
  Zero-Order Hold : ZeroOrderHold  SampleTime=Ts(2)
  epsilon : Scope
  Tt_corrected : Outport
  wires:
  Bus Selector2/11 -> MATLAB Function/11("theta_s_dot ")  "<theta_s_dot_R_L>"
  RL_weights/1(exponents) -> Subsystem1/1(exponents)
  ROAD PREVIEW/1(Online Data) -> Rule based/1(Online Data), Rate Transition4/1, RL_weights/2(Online Data)  "Online Data"
  Constant1/1 -> Rate Transition6/1  "Number of iterations"
  MATLAB Function/8(x_u_R_L) -> Bus Creator1/8  "x_u_R_L"
  Constant2/1 -> Multiport Switch1/1, Multiport Switch3/1
  Bus Selector2/6 -> MATLAB Function/6(x_b)  "<x_b>"
  MATLAB Function/2(z_b_R) -> Bus Creator1/2  "z_b_R"
  Subsystem2/1(stage cost matrix) -> Multiport Switch3/4
  Subsystem1/1(stage cost matrix) -> Multiport Switch3/3
  MATLAB Function/3(z_u_dot_R_L) -> Bus Creator1/3  "z_u_dot_R_L"
  Rule based/1(exponents) -> Subsystem2/1(exponents)
  Bus Selector2/4 -> MATLAB Function/4("z_u_R_L ")  "<z_u_R_L>"
  Constant/1 -> MATLAB Function/16(b)
  Rate Transition2/1 -> Longitudinal_Vibration_NMPC_UoS/3
  Rate Transition4/1 -> Longitudinal_Vibration_NMPC_UoS/6
  Multiport Switch1/1 -> Rate Transition3/1  "Terminal Cost Matrix"
  Longitudinal_Vibration_NMPC_UoS/5 -> Terminator3/1  "KKT optimization tolerance"
  Bus Selector2/15 -> MATLAB Function/15(pitch)  "<pitch>"
  Bus Selector2/1 -> MATLAB Function/1(z_b_dot)  "<z_b_dot>"
  Bus Selector2/8 -> MATLAB Function/8("x_u_R_L ")  "<x_u_R_L>"
  Bus Selector2/2 -> MATLAB Function/2(z_b)  "<z_b>"
  Demux/1 -> Saturation/1
  MATLAB Function/10(theta_w) -> Bus Creator1/10  "theta_w"
  MATLAB Function/11(theta_s_dot) -> Bus Creator1/11  "theta_s_dot"
  Bus Selector2/9 -> MATLAB Function/9("theta_w_dot ")  "<omega_R_L>"
  Longitudinal_Vibration_NMPC_UoS/6 -> Terminator2/1  "(no timing)"
  Longitudinal_Vibration_NMPC_UoS/2 -> Terminator6/1  "States prediction"
  Bus Selector2/7 -> MATLAB Function/7("x_u_dot_R_L ")  "<x_u_dot_R_L>"
  Longitudinal_Vibration_NMPC_UoS/7 -> Terminator1/1
  MATLAB Function/9(theta_w_dot) -> Bus Creator1/9  "theta_w_dot"
  Demux/2 -> epsilon/1  "epsilon"
  MATLAB Function/13(torque) -> Bus Creator1/13  "torque"
  Longitudinal_Vibration_NMPC_UoS/3 -> Terminator5/1  "Control Inputs Prediction"
  Bus Selector2/10 -> MATLAB Function/10("theta_w ")  "<theta_R_L>"
  Subsystem1/2(terminal cost matrix) -> Multiport Switch1/3
  Longitudinal_Vibration_NMPC_UoS/8 -> Integrator/1  "NMPC Objective Value"
  BUS/1 -> Rule based/2(BUS), ROAD PREVIEW/2(CAN), RL_weights/1(States), Bus Selector1/1, Bus Selector2/1
  MATLAB Function/12(theta_s) -> Bus Creator1/12  "theta_s"
  Bus Selector2/17 -> Reference acceleration/3(Ft2)  "<Ft_F_req>"
  Ground1/1 -> Rate Transition5/1  "Constraints"
  Rate Transition5/1 -> Longitudinal_Vibration_NMPC_UoS/5
  Bus Selector2/5 -> MATLAB Function/5(x_b_dot)  "<x_b_dot>"
  MATLAB Function/4(z_u_R_L) -> Bus Creator1/4  "z_u_R_L"
  Bus Selector2/16 -> Reference acceleration/1(Ft), ROAD PREVIEW/1(F_t)  "<Ft_R_req>"
  MATLAB Function/5(x_b_dot_R) -> Bus Creator1/5  "x_b_dot_R"
  Bus Selector2/14 -> MATLAB Function/14(pitch_dot)  "<pitch_dot>"
  MATLAB Function/6(x_b_R) -> Bus Creator1/6  "x_b_R"
  Integrator/1 -> Terminator4/1
  Bus Selector2/13 -> MATLAB Function/13("torque ")  "<Tm_R_L>"
  MATLAB Function/7(x_u_dot_R_L) -> Bus Creator1/7  "x_u_dot_R_L"
  Rate Transition3/1 -> Longitudinal_Vibration_NMPC_UoS/4
  Bus Selector2/3 -> MATLAB Function/3("z_u_dot_R_L ")  "<z_u_dot_R_L>"
  MATLAB Function/1(z_b_dot_R) -> Bus Creator1/1  "z_b_dot_R"
  Rate Transition6/1 -> Longitudinal_Vibration_NMPC_UoS/7
  Saturation/1 -> Tt_corrected/1
  Weight matrixes/1(Stage Cost Matrix) -> Multiport Switch3/2  "Stage Cost Matrix"
  Bus Selector/1 -> Reference acceleration/2(x_b_dot)  "<x_b_dot_R>"
  Rate Transition1/1 -> Longitudinal_Vibration_NMPC_UoS/2
  Bus Selector2/12 -> MATLAB Function/12("theta_s ")  "<theta_s_R_L>"
  Rate Transition/1 -> Longitudinal_Vibration_NMPC_UoS/1
  Longitudinal_Vibration_NMPC_UoS/4 -> Solver status RL/1  "Status QP Solver"
  Bus Creator1/1 -> Rate Transition/1, Bus Selector/1  "States"
  Weight matrixes/2(Terminal Cost Matrix) -> Multiport Switch1/2  "Terminal Cost Matrix"
  Subsystem2/2(terminal cost matrix) -> Multiport Switch1/4
  Longitudinal_Vibration_NMPC_UoS/1 -> Zero-Order Hold/1  "First Control Input"
  Zero-Order Hold/1 -> Demux/1
  Bus Selector1/1 -> Weight matrixes/1(x_u)  "<x_u_R_L>"
  Reference acceleration/1(a_ref) -> Reference Generation/1(a_b_ref), RL_weights/3(a_b_ref)
  Reference Generation/1(References) -> Rate Transition1/1  "References"
  MATLAB Function1/1(cost_fcn_weights) -> To Workspace9/1
  Multiport Switch3/1 -> Rate Transition2/1, MATLAB Function1/1(Wmat_NMPC)  "Stage Cost Matrix"

== system Full_Car_Model/CONTROLLER REAR RIGHT ==
  BUS : Inport
  Bus Creator1 : BusCreator  Inputs=13
  Bus Selector : BusSelector  OutputSignals=x_b_dot_R
  Bus Selector1 : BusSelector  OutputSignals=States.x_u_R_R
  Bus Selector2 : BusSelector  OutputSignals=States.z_b_dot,States.z_b,States.z_u_dot_R_R,States.z_u_R_R,States.x_b_dot,States.x_b,States.x_u_dot_R_R,States.x_u_R_R,States.omega_R_R,States.theta_R_R,Differentials.theta_s_dot_R_R,Differentials.theta_s_R_R,Traction_forces.Tm_R_R,States.pitch_dot,States.pitch,Traction_forces.Ft_R_req,Traction_forces.Ft_F_req
  Constant : Constant  Value=data.b
  Constant1 : Constant  Value=N_iter
  Constant2 : Constant  Value=adaptive
  Demux : Demux  Outputs=2
  Ground1 : Ground
  Integrator : Integrator
  Longitudinal_Vibration_NMPC_UoS : S-Function  FunctionName=acado_solver_sfun_NMPC_RR  Parameters=xInit, zInit, uInit, Wmat_NMPC_init, WNmat_NMPC_init, bValues  SFunctionDeploymentMode=off  EnableBusSupport=off  mask(Legacy Function){SFunctionSpec=acado_step(ACADOinput u1[1], ACADOoutput y1[1]), ShowSpec=on}
      mask prompts: ShowSpec "Display function specification"
      mask help:
      | This block allows you to call the legacy functions specified by the following Legacy Code Tool definition:
      | def.SFunctionName = 'acado_solver_sfun';
      | def.OutputFcnSpec = 'acado_step(ACADOinput u1[1], ACADOoutput y1[1])';
      | def.StartFcnSpec = 'acado_initialize( void )';
      | def.TerminateFcnSpec = 'acado_cleanup( void )';
      | def.HeaderFiles = {'acado_common.h', 'acado_solver_sfunction.h'};
      | def.SourceFiles = {'acado_solver.c', 'acado_integrator.c', 'acado_auxiliary_functions.c', 'acado_solver_sfunction.c', 'acado_qpoases_interface.cpp', 'qpoases/SRC/Bounds.cpp', 'qpoases/SRC/Constraints.cpp', 'qpoases/SRC/CyclingManager.cpp', 'qpoases/SRC/Indexlist.cpp', 'qpoases/SRC/MessageHandling.cpp', 'qpoases/SRC/QProblem.cpp', 'qpoases/SRC/QProblemB.cpp', 'qpoases/SRC/SubjectTo.cpp', 'qpoases/SRC/Utils.cpp', 'qpoases/SRC/EXTRAS/SolutionAnalysis.cpp'};
      | def.IncPaths = {'qpoases', 'qpoases/INCLUDE', 'qpoases/SRC'};
      | def.Options.language = 'C++';
      mask Help: <p>This block was generated automatically by the Legacy Code Tool. For detailed help on this tool, call<a href="matlab:legacy_code('help')"> legacy_code('help')</a>.</p>
      mask Callback ShowSpec:
      | if strcmp(get_param(gcbh, 'ShowSpec'), 'on')
      |   set_param(gcbh, 'MaskDisplay', sprintf('fprintf(''%s'');', get_param(gcbh, 'SFunctionSpec')));
      | else
      |   set_param(gcbh, 'MaskDisplay', sprintf('fprintf(''%s'');', get_param(gcbh, 'FunctionName')));
      | end
      mask Display: fprintf('acado_step(ACADOinput u1[1], ACADOoutput y1[1])');
  MATLAB Function : MATLAB Function  TreatAsAtomicUnit=on
  Multiport Switch1 : MultiPortSwitch  SaturateOnIntegerOverflow=off  InputSameDT=off
  Multiport Switch3 : MultiPortSwitch  SaturateOnIntegerOverflow=off  InputSameDT=off
  RL_weights : Subsystem
  ROAD PREVIEW : Subsystem
  Rate Transition : RateTransition  InitialCondition=X_0  OutPortSampleTime=Ts(2)
  Rate Transition{1,4..6} (4 alike) : RateTransition  OutPortSampleTime=Ts(2)
  Rate Transition2 : RateTransition  InitialCondition=Wmat_NMPC_init  OutPortSampleTime=Ts(2)
  Rate Transition3 : RateTransition  InitialCondition=WNmat_NMPC_init  OutPortSampleTime=Ts(2)
  Reference Generation : MATLAB Function  TreatAsAtomicUnit=on
  Reference acceleration : Subsystem
  Rule based : Subsystem
  Saturation : Saturate  UpperLimit=data.Ub_Tm  LowerLimit=data.Lb_Tm
  Subsystem1 : Subsystem
  Subsystem2 : Subsystem
  Terminator{1..8} (8 alike) : Terminator
  Weight matrixes : Subsystem
  Zero-Order Hold : ZeroOrderHold  SampleTime=Ts(2)
  Tt_corrected : Outport
  wires:
  RL_weights/1(exponents) -> Subsystem1/1(exponents)
  Demux/2 -> Terminator8/1  "epsilon"
  ROAD PREVIEW/1(Online Data) -> Rule based/1(Online Data), Rate Transition4/1, RL_weights/2(Online Data)  "Online Data"
  Multiport Switch3/1 -> Rate Transition2/1  "Stage Cost Matrix"
  Bus Selector2/16 -> Reference acceleration/1(Ft), ROAD PREVIEW/1(F_t)  "<Ft_R_req>"
  Longitudinal_Vibration_NMPC_UoS/7 -> Terminator1/1
  Bus Creator1/1 -> Rate Transition/1, Bus Selector/1  "States"
  Rule based/1(exponents) -> Subsystem2/1(exponents)
  MATLAB Function/10(theta_w) -> Bus Creator1/10  "theta_w"
  Subsystem2/2(terminal cost matrix) -> Multiport Switch1/4
  Bus Selector2/9 -> MATLAB Function/9("theta_w_dot ")  "<omega_R_R>"
  Longitudinal_Vibration_NMPC_UoS/5 -> Terminator3/1  "KKT optimization tolerance"
  MATLAB Function/5(x_b_dot_R) -> Bus Creator1/5  "x_b_dot_R"
  Rate Transition4/1 -> Longitudinal_Vibration_NMPC_UoS/6
  Subsystem2/1(stage cost matrix) -> Multiport Switch3/4
  Rate Transition2/1 -> Longitudinal_Vibration_NMPC_UoS/3
  MATLAB Function/13(torque) -> Bus Creator1/13  "torque"
  Ground1/1 -> Rate Transition5/1  "Constraints"
  Subsystem1/1(stage cost matrix) -> Multiport Switch3/3
  Reference Generation/1(References) -> Rate Transition1/1  "References"
  MATLAB Function/12(theta_s) -> Bus Creator1/12  "theta_s"
  MATLAB Function/9(theta_w_dot) -> Bus Creator1/9  "theta_w_dot"
  Rate Transition6/1 -> Longitudinal_Vibration_NMPC_UoS/7
  Constant2/1 -> Multiport Switch1/1, Multiport Switch3/1
  Weight matrixes/2(Terminal Cost Matrix) -> Multiport Switch1/2  "Terminal Cost Matrix"
  Bus Selector2/8 -> MATLAB Function/8("x_u_R_R ")  "<x_u_R_R>"
  Bus Selector2/6 -> MATLAB Function/6(x_b)  "<x_b>"
  MATLAB Function/7(x_u_dot_R_R) -> Bus Creator1/7  "x_u_dot_R_R"
  MATLAB Function/8(x_u_R_R) -> Bus Creator1/8  "x_u_R_R"
  Bus Selector2/15 -> MATLAB Function/15(pitch)  "<pitch>"
  MATLAB Function/11(theta_s_dot) -> Bus Creator1/11  "theta_s_dot"
  Bus Selector2/4 -> MATLAB Function/4("z_u_R_R ")  "<z_u_R_R>"
  Longitudinal_Vibration_NMPC_UoS/3 -> Terminator5/1  "Control Inputs Prediction"
  Weight matrixes/1(Stage Cost Matrix) -> Multiport Switch3/2  "Stage Cost Matrix"
  Bus Selector2/2 -> MATLAB Function/2(z_b)  "<z_b>"
  Bus Selector2/3 -> MATLAB Function/3("z_u_dot_R_R ")  "<z_u_dot_R_R>"
  MATLAB Function/2(z_b_R) -> Bus Creator1/2  "z_b_R"
  BUS/1 -> Rule based/2(BUS), ROAD PREVIEW/2(CAN), RL_weights/1(States), Bus Selector1/1, Bus Selector2/1
  MATLAB Function/6(x_b_R) -> Bus Creator1/6  "x_b_R"
  Bus Selector2/7 -> MATLAB Function/7("x_u_dot_R_R ")  "<x_u_dot_R_R>"
  Longitudinal_Vibration_NMPC_UoS/6 -> Terminator4/1  "(no timing)"
  Rate Transition/1 -> Longitudinal_Vibration_NMPC_UoS/1
  Bus Selector2/17 -> Reference acceleration/3(Ft2)  "<Ft_F_req>"
  Longitudinal_Vibration_NMPC_UoS/2 -> Terminator6/1  "States prediction"
  Bus Selector/1 -> Reference acceleration/2(x_b_dot)  "<x_b_dot_R>"
  Constant1/1 -> Rate Transition6/1  "Number of iterations"
  Bus Selector2/10 -> MATLAB Function/10("theta_w ")  "<theta_R_R>"
  MATLAB Function/4(z_u_R_R) -> Bus Creator1/4  "z_u_R_R"
  Rate Transition3/1 -> Longitudinal_Vibration_NMPC_UoS/4
  Bus Selector2/11 -> MATLAB Function/11("theta_s_dot ")  "<theta_s_dot_R_R>"
  Bus Selector2/13 -> MATLAB Function/13("torque ")  "<Tm_R_R>"
  Bus Selector2/1 -> MATLAB Function/1(z_b_dot)  "<z_b_dot>"
  Longitudinal_Vibration_NMPC_UoS/8 -> Integrator/1  "NMPC Objective Value"
  Integrator/1 -> Terminator7/1
  Bus Selector2/5 -> MATLAB Function/5(x_b_dot)  "<x_b_dot>"
  Rate Transition5/1 -> Longitudinal_Vibration_NMPC_UoS/5
  MATLAB Function/1(z_b_dot_R) -> Bus Creator1/1  "z_b_dot_R"
  Saturation/1 -> Tt_corrected/1
  Bus Selector2/12 -> MATLAB Function/12("theta_s ")  "<theta_s_R_R>"
  MATLAB Function/3(z_u_dot_R_R) -> Bus Creator1/3  "z_u_dot_R_R"
  Rate Transition1/1 -> Longitudinal_Vibration_NMPC_UoS/2
  Constant/1 -> MATLAB Function/16(b)
  Longitudinal_Vibration_NMPC_UoS/4 -> Terminator2/1  "Status QP Solver"
  Multiport Switch1/1 -> Rate Transition3/1  "Terminal Cost Matrix"
  Bus Selector2/14 -> MATLAB Function/14(pitch_dot)  "<pitch_dot>"
  Subsystem1/2(terminal cost matrix) -> Multiport Switch1/3
  Longitudinal_Vibration_NMPC_UoS/1 -> Zero-Order Hold/1  "First Control Input"
  Demux/1 -> Saturation/1
  Zero-Order Hold/1 -> Demux/1
  Bus Selector1/1 -> Weight matrixes/1(x_u)  "<x_u_R_R>"
  Reference acceleration/1(a_ref) -> RL_weights/3(a_b_ref), Reference Generation/1(a_b_ref)

== system Full_Car_Model/NMPC Internal model FL ==
  BUS : Inport
  1-D Lookup Table2 : Lookup_n-D  NumberOfTableDimensions=1  BreakpointsForDimension1=mu_distance  Table=mu_road  InternalRulePriority=Speed  RndMeth=Simplest
  Bus Creator : BusCreator  Inputs=6
  Bus Creator1 : BusCreator  Inputs=3
  Bus Creator2 : BusCreator  Inputs=3
  Bus Creator3 : BusCreator  Inputs=6
  Bus Creator5 : BusCreator  Inputs=4
  Bus Selector : BusSelector  OutputSignals=Traction_forces.Tm_F_L,Traction_forces.Ft_F_req,Traction_forces.Ft_R_req,Accelerations.x_b_ddot,States.z_u_dot_F_L,States.z_u_F_L,Accelerations.z_u_ddot_F_L
  Bus Selector1 : BusSelector  OutputSignals=Horizontal.x_b_dot,Horizontal.x_b,Horizontal.x_u_dot,Horizontal.x_u,Vertical.z_b_dot,Vertical.z_b,Vertical.z_u_dot,Vertical.z_u,Rotational.theta_w_dot,Rotational.theta_w,Half Shaft.theta_s_dot,Half Shaft.theta_s
  Bus Selector2 : BusSelector  OutputSignals=Vertical.z_u,Vertical.z_u_dot,Vertical.z_u_ddot,Horizontal.x_b_ddot
  Integrator1 : Integrator  InitialCondition=z_u_dot_ini_F_L
  Integrator10 : Integrator  InitialCondition=x_b_dot_ini
  Integrator11 : Integrator  InitialCondition=x_b_ini + data.a
  Integrator12 : Integrator  InitialCondition=theta_s_ini_F_L
  Integrator2 : Integrator  InitialCondition=z_u_ini_F_L
  Integrator3 : Integrator  InitialCondition=x_u_dot_ini_F_L
  Integrator4 : Integrator  InitialCondition=z_b_dot_ini
  Integrator5 : Integrator  InitialCondition=z_b_ini
  Integrator6 : Integrator  InitialCondition=omega_ini_F_L
  Integrator7 : Integrator
  Integrator8 : Integrator  InitialCondition=x_u_ini_F_L
  Integrator9 : Integrator  InitialCondition=omega_ini_F_L
  MATLAB Function1 : MATLAB Function  TreatAsAtomicUnit=on
  Multiply : Gain  Gain=data.R_F
  Multiply1 : Gain  Gain=data.R_R
  Multiply2 : Gain  Gain=1500/data.Tm_max
  Multiply3 : Gain  Gain=1500/data.Tm_max
  Mux : Mux  Inputs=13
  Mux1 : Mux  Inputs=2
  Product : Product
  Product1 : Product
  Scope{,1..3} (4 alike) : Scope  NumInputPorts=2
  Time-based Road Preview : Subsystem
  To Workspace : ToWorkspace  VariableName=x_b_ddot_pred  SaveFormat=Timeseries  SampleTime=-1
  wires:
  Bus Selector/4 -> Scope/2  "<x_b_ddot>"
  Bus Selector2/4 -> To Workspace/1, Scope/1  "<x_b_ddot>"
  Bus Selector1/1 -> Mux/1  "<x_b_dot>"
  Bus Selector1/2 -> Mux/2  "<x_b>"
  MATLAB Function1/4(x_u_ddot) -> Integrator3/1, Bus Creator3/6  "x_u_ddot"
  Bus Selector1/4 -> 1-D Lookup Table2/1, Time-based Road Preview/1(x_u), Mux/4  "<x_u>"
  Bus Selector1/3 -> Mux/3  "<x_u_dot>"
  Mux/1 -> MATLAB Function1/1(States)
  Integrator8/1 -> Bus Creator3/4  "x_u"
  MATLAB Function1/1(z_b_ddot) -> Integrator4/1, Bus Creator/3  "z_b_ddot"
  MATLAB Function1/3(x_b_ddot) -> Integrator10/1, Bus Creator3/3  "x_b_ddot"
  Bus Selector1/8 -> Mux/8  "<z_u>"
  Integrator6/1 -> Bus Creator2/2, Integrator7/1  "theta_w_dot"
  Integrator10/1 -> Bus Creator3/2, Integrator11/1  "x_b_dot"
  Integrator11/1 -> Bus Creator3/1  "x_b"
  MATLAB Function1/5(theta_w_ddot) -> Integrator6/1, Bus Creator2/3  "theta_w_ddot"
  Bus Creator/1 -> Bus Creator5/1  "Vertical"
  Bus Selector1/5 -> Mux/5  "<z_b_dot>"
  Bus Selector1/10 -> Mux/10  "<theta_w>"
  Bus Selector1/6 -> Mux/6  "<z_b>"
  Integrator5/1 -> Bus Creator/1  "z_b"
  Integrator4/1 -> Bus Creator/2, Integrator5/1  "z_b_dot"
  Integrator2/1 -> Bus Creator/4  "z_u"
  Bus Creator5/1 -> Bus Selector1/1, Bus Selector2/1
  Bus Selector1/7 -> Mux/7  "<z_u_dot>"
  Integrator1/1 -> Bus Creator/5, Integrator2/1  "z_u_dot"
  Bus Creator3/1 -> Bus Creator5/2  "Horizontal"
  Integrator3/1 -> Bus Creator3/5, Integrator8/1  "x_u_dot"
  MATLAB Function1/2(z_u_ddot) -> Integrator1/1, Bus Creator/6  "z_u_ddot"
  Bus Selector/2 -> Multiply/1  "<Ft_F_req>"
  BUS/1 -> Bus Selector/1
  Time-based Road Preview/1(w) -> Mux1/1
  Time-based Road Preview/2(beta_y) -> Mux1/2
  Bus Creator2/1 -> Bus Creator5/3  "Rotational"
  Bus Selector/3 -> Multiply1/1  "<Ft_R_req>"
  Multiply/1 -> Multiply3/1
  Integrator7/1 -> Bus Creator2/1  "theta_w"
  Integrator9/1 -> Bus Creator1/2, Integrator12/1  "theta_s_dot"
  MATLAB Function1/6(theta_s_ddot) -> Integrator9/1, Bus Creator1/3  "theta_s_ddot"
  Bus Creator1/1 -> Bus Creator5/4  "Half Shaft"
  Integrator12/1 -> Bus Creator1/1  "theta_s"
  Bus Selector1/9 -> Mux/9  "<theta_w_dot>"
  Bus Selector1/11 -> Mux/11  "<theta_s_dot>"
  Bus Selector1/12 -> Mux/12  "<theta_s>"
  Multiply3/1 -> Product/1  "Tm_req_F2"
  Multiply2/1 -> Product1/1
  Multiply1/1 -> Multiply2/1
  Bus Selector/1 -> Mux/13  "<Tm_F_L>"
  Mux1/1 -> MATLAB Function1/2(road)
  1-D Lookup Table2/1 -> MATLAB Function1/6(mu_act)
  Product/1 -> MATLAB Function1/3(Tm_req_F2)
  Product1/1 -> MATLAB Function1/4(Tm_req_R_L), MATLAB Function1/5(Tm_req_R_R)
  Bus Selector2/1 -> Scope1/1  "<z_u>"
  Bus Selector2/2 -> Scope2/1  "<z_u_dot>"
  Bus Selector/5 -> Scope2/2  "<z_u_dot_F_L>"
  Bus Selector/6 -> Scope1/2  "<z_u_F_L>"
  Bus Selector2/3 -> Scope3/1  "<z_u_ddot>"
  Bus Selector/7 -> Scope3/2  "<z_u_ddot_F_L>"
  [mu_swift_F_L] -> Product/2
  [mu_swift_R_L] -> Product1/2
